simulink model "reachout_demo_PERTURB_EP_2010a"  (Simulink 7.5)
settings: Solver=ode4  SolverMode=SingleTasking  StartTime=0.0  StopTime=inf  FixedStep=0.0005  RelTol=1e-3
model workspace (MAT data in the model file):
  col_x = 1
  col_y = 2
  RADIUS_VIS = 3
  RADIUS_LOG = 4
  COLOR_INIT = 5
  COLOR_REACH = 6
  START_TARGET_COL = 1
  END_TARGET_COL = 2
  LOAD_COL = 3
  DELAY_HAND_FDBK_ON_COL = 4
  MAXREACHTIME_COL = 7
  DELAY_POSTTRIAL_COL = 9
  HAND_FDBK_CNTL_COL = 10
  E_STAY_CENTER = 2
  E_TARGET_ON = 3
  E_HOLD_AT_TARGET = 5
  E_HAND_FDBK_ON = 10
  E_HAND_FDBK_OFF = 11
  WAIT_AT_1stTARGET_COL = 5
  RNDM_WAIT_AT_1stTARGET_COL = 6
  WAIT_AT_2ndTARGET_COL = 8
  X_COL = 1
  Y_COL = 2
  RISE_FALL_COL = 3
  DURATION_COL = 4
StartFcn:
  |  warndlg('Dexterit-E models cannot run under simulation. Please compile your model and run it from within Dexterit-E.');set_param(bdroot,'SimulationCommand','stop')
libraries: General x3, Video x3, KINARM_EP_loads x2, KINARM_general x2, KINARM_loads x1
CloseFcn:
  | rtwprivate ssgencode ModelCloseRequest b2lab2d
settings Model: Creator=Chris Grebeldinger  LastModifiedBy=BKIN TECHNOLOGIES  ModifiedComment=chris -- Wed Feb 16 09:18:30 2005 -- Version 1.1384  ModifiedHistory=Feb 16/05 - Add error repeat, add offset ramp  ExtModeArmWhenConnect=off  ExtModeLogAll=off  BufferReuse=off
settings DataIOCC: LimitDataPoints=off  SaveOutput=off  SaveTime=off  SignalLoggingName=sigsOut
settings OptimizationCC: BlockReduction=off  BooleanDataType=off  OptimizeBlockIOStorage=off  BufferReuse=off  ExpressionFolding=off  FoldNonRolledExpr=off  LocalBlockOutputs=off  InitFltsAndDblsToZero=on
settings DebuggingCC: SaveWithParameterizedLinksMsg=none  SignalResolutionControl=TryResolveAllWithWarning  SolverPrmCheckMsg=none  MultiTaskDSMMsg=warning  MultiTaskCondExecSysMsg=none  StrictBusMsg=None
settings HardwareCC: ProdIntDivRoundTo=Zero  ProdEndianess=LittleEndian  ProdHWDeviceType=Generic->32-bit x86 compatible  TargetHWDeviceType=32-bit Generic
settings RTWCC: SystemTargetFile=xpctarget.tlc  TemplateMakefile=xpc_default_tmf  Description=xPC Target  ProcessScript=xpctarget_make_rtw_hook  IncludeERTFirstTime=on  RTWCompilerOptimization=On
settings CodeAppCC: MaxIdLength=63  CustomSymbolStrType=$N$R$M_T
settings xpcTargetCC: TargetFcnLib=ansi_tfl_tmw.mat  TargetFunctionLibrary=ANSI_C  ParMdlRefBuildCompliant=on  ConcurrentExecutionCompliant=on  CombineSignalStateStructs=off  GRTInterface=on  GenerateAllocFcn=off  xPCTaskExecutionProfile=off  xPCRL32EventNumber=5000  xPCisDownloadable=off  xPCLoadParamSetFile=off  xPCConcurrentTasks=off  xPCEnableSFAnimation=off

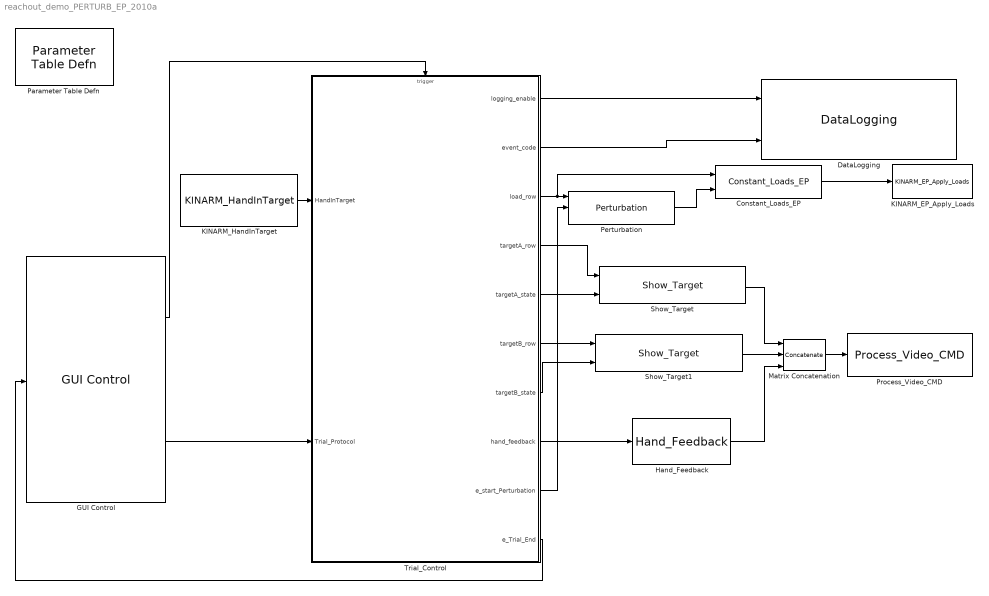
== system reachout_demo_PERTURB_EP_2010a ==
  Constant_Loads_EP : KINARM_EP_loads/Constant_Loads_EP  use_dom_hand=on  loadcol="[1  2]"  source=external  scaling=1  use_LH_coord=off
  DataLogging : General/DataLogging  log_event_codes=on  log_analog_inputs=off
      link override Poll KINARM/EPTorqueCMD: GotoTag=KINARMEPTorqueCMD
  GUI Control : General/GUI Control  target_type_str=Circle  Target_Type=1  XYcols=[1 2]  Vcols=3  Lcols=4  indices_padding=[0 0 0 0;0 0 0 0]  task_version=1.0  show_repeat_trial_flag=off
  Hand_Feedback : KINARM_general/Hand_Feedback  feedback_cntl_src=status only
  KINARM_EP_Apply_Loads : KINARM_EP_loads/KINARM_EP_Apply_Loads  up_duration=1500  down_duration=1500  max_force=60
  KINARM_HandInTarget : KINARM_general/KINARM_HandInTarget  use_dominant_hand=on  target_type=Circle  num_states=1  attribcol1=4  attribcol2=4  attribcol3=5  attribcol4=6
  Matrix Concatenation : Concatenate  NumInputs=3  Mode=Multidimensional array
  Parameter Table Defn : General/Parameter Table Defn  ShowInLibBrowser=0
  Perturbation : KINARM_loads/Perturbation  loadcol="[3  4  3]"
  Process_Video_CMD : Video/Process_Video_CMD
  Show_Target : Video/Show_Target  target_type=Circle  num_states=2  attribcol1=[5 5 0 3]  attribcol2=[6 6 0 3]  attribcol3=[0 0 0 0]  attribcol4=[0 0 0 0]  attribcol5=[0 0 24 0]  stateindices_padding=[0 0 0 0 0 0 0;0 0 0 0 0 0 0;0 0 0 0 0 0 0;0 0 0 0 0 0 0;0 0 0 0 0 0 0]  source=internal  opacity=100  target_display=Both subject and operator displays
  Show_Target1 : Video/Show_Target  target_type=Circle  num_states=2  attribcol1=[5 5 0 3]  attribcol2=[6 6 0 3]  attribcol3=[0 0 0 0]  attribcol4=[0 0 0 0]  attribcol5=[0 0 24 0]  stateindices_padding=[0 0 0 0 0 0 0;0 0 0 0 0 0 0;0 0 0 0 0 0 0;0 0 0 0 0 0 0;0 0 0 0 0 0 0]  source=internal  opacity=100  target_display=Both subject and operator displays
  Trial_Control : Stateflow chart  TreatAsAtomicUnit=on
      settings: PermitHierarchicalResolution=ParametersOnly
  wires:
  KINARM_HandInTarget/1 -> Trial_Control/1(HandInTarget)
  Show_Target/1 -> Matrix Concatenation/1
  GUI Control/2 -> Trial_Control/2(Trial_Protocol)
  Trial_Control/10(e_Trial_End) -> GUI Control/1
  GUI Control/1 -> Trial_Control/Trigger
  Trial_Control/5(targetA_state) -> Show_Target/2
  Trial_Control/4(targetA_row) -> Show_Target/1
  Matrix Concatenation/1 -> Process_Video_CMD/1
  Trial_Control/8(hand_feedback) -> Hand_Feedback/1
  Hand_Feedback/1 -> Matrix Concatenation/3
  Show_Target1/1 -> Matrix Concatenation/2
  Trial_Control/6(targetB_row) -> Show_Target1/1
  Trial_Control/7(targetB_state) -> Show_Target1/2
  Constant_Loads_EP/1 -> KINARM_EP_Apply_Loads/1
  Trial_Control/3(load_row) -> Perturbation/1, Constant_Loads_EP/1
  Perturbation/1 -> Constant_Loads_EP/2
  Trial_Control/9(e_start_Perturbation) -> Perturbation/2
  Trial_Control/1(logging_enable) -> DataLogging/1
  Trial_Control/2(event_code) -> DataLogging/2

== stateflow chart Trial_Control ==
  settings: sampleTime=0.001
  state Inter_Trial_State/
    // send e_Trial_End event
    e_Trial_End;
    // turn off both targets
    // stop data logging
    targetA_state=0;
    targetB_state=0;
    logging_enable = 0;
  state Main_Trial
    state Show2ndTarget/
      // Turn on second target, log an event, wait until hand-is-in-target or for specified delay
      event_code=E_TARGET_ON;
      targetB_row = Trial_Protocol[END_TARGET_COL];
      targetB_state=1;
      tickCount =Trial_Protocol[MAXREACHTIME_COL];
      e_start_Perturbation;
    state StayAt2ndTarget/
      // change the 2nd target's state, log an event, wait for a specified period of time
      event_code=E_HOLD_AT_TARGET;
      targetB_state=2;
      tickCount =Trial_Protocol[WAIT_AT_2ndTARGET_COL];
    state EndOfTrial/
      // Wait for a specified period of time,
      tickCount =Trial_Protocol[DELAY_POSTTRIAL_COL];
    state StayAtFirstTarget/
      // change the first target state, log an event, wait for specified (randomized) period of time.  Hand must STAY in target for specified time.
      logging_enable = 1;
      event_code=E_STAY_CENTER
      targetA_state=2;
      tickCount =Trial_Protocol[WAIT_AT_1stTARGET_COL]+Trial_Protocol[RNDM_WAIT_AT_1stTARGET_COL]*rand()/RAND_MAX;
    state FirstTargetOn/
      // Turn on first target, set loading conditions, enable data logging, wait for specified delay or until hand-is-in-target
      targetA_row = Trial_Protocol[START_TARGET_COL];
      targetA_state=1;
      load_row = Trial_Protocol[LOAD_COL];
      tickCount =Trial_Protocol[DELAY_HAND_FDBK_ON_COL]
    state HandFeedbackOn/
      // Turn on handfeedback
      hand_feedback=1;
    state WaitOneStep/
      // Delay one step for E_HAND_FEEDBACK_OFF to
      // be processed prior to next state
    FirstTargetOn -> HandFeedbackOn [order 2] : [HandInTarget[targetA_row]==1]
    FirstTargetOn -> HandFeedbackOn [order 1] : after(tickCount, e_clk)
    StayAtFirstTarget -> HandFeedbackOn [order 2] : [HandInTarget[targetA_row]==0]
    HandFeedbackOn -> StayAtFirstTarget : [HandInTarget[targetA_row]==1]
    StayAtFirstTarget -> (junction 13) [order 1] : after(tickCount, e_clk)
        | {hand_feedback=Trial_Protocol[HAND_FDBK_CNTL_COL]}
        | // Turn handfeedback on or off (from Trial Protocol Table)
    (junction 13) -> WaitOneStep [order 2]
    (junction 13) -> WaitOneStep [order 1] : [hand_feedback==0]/
        | // if hand feedback is turned off, log an event
        | event_code=E_HAND_FDBK_OFF;
    WaitOneStep -> Show2ndTarget
    Show2ndTarget -> StayAt2ndTarget [order 2] : [HandInTarget[targetB_row]==1]
    Show2ndTarget -> EndOfTrial [order 1] : after(tickCount, e_clk)/
    StayAt2ndTarget -> EndOfTrial : after(tickCount, e_clk)
  state Initialize/
    // Turn off both targets, set hand_feedback on
    targetA_state=0;
    targetB_state=0;
    hand_feedback=1;
  (default) -> Initialize
  Initialize -> FirstTargetOn
  Inter_Trial_State -> FirstTargetOn : after(tickCount, e_clk)
  Main_Trial -> Inter_Trial_State : e_ExitTrialNow/
      | // if e_ExitTrialNow event occurs,
      | tickCount=1;
  EndOfTrial -> Inter_Trial_State
  data: HandInTarget input double; logging_enable output boolean; event_code output uint16 [0..] =0; load_row output double [1..32]; Trial_Protocol input double; targetA_row output double [1..32]; targetA_state output double; targetB_row output double; targetB_state output double; tickCount local double; hand_feedback output double; RAND_MAX constant double =32767
  data load_row settings: description=current index into the loadtable
  data targetA_row settings: description=index of the row currently being used in the TargetTable
  events: e_start_Perturbation output EITHER_EDGE_EVENT; e_clk input RISING_EDGE_EVENT; e_ExitTrialNow input EITHER_EDGE_EVENT; e_Trial_End output EITHER_EDGE_EVENT
